simulink model "ATOM_simple_planning_simulator"  (R2026a)
settings: Solver=ode4  StopTime=100  FixedStep=0.01
StopFcn:
  | % Put every new figure in the same MATLAB Figures window as a docked tab.
  | set(groot, 'defaultFigureWindowStyle', 'docked');
  | 
  | if exist('costmap_active', 'var') && ...
  |     exist('vehicle', 'var') && ...
  |     exist('parking_path', 'var') && ...
  |     ~isempty(parking_path)
  | 
  |      plotPlan(costmap_active, vehicle, parking_path);
  | 
  |  else
  | 
  |      warning('No valid parking path is available for plotting.');
  | 
  |  end
  | 
  |  PlotControllerReferences( ...
  |      out.controller_reference_log);
  | 
  |  PlotControllerTracking( ...
  |      out.controller_tracking_log);
  | 
model workspace (MAT data in the model file):
  vehicle.param.wheel_radius = 0.313
  vehicle.param.wheel_width = 0.235
  vehicle.param.wheel_base = 2
  vehicle.param.wheel_tread = 1.9
  vehicle.param.front_overhang = 0.46
  vehicle.param.rear_overhang = 0.46
  vehicle.param.left_overhang = 0.128
  vehicle.param.right_overhang = 0.128
  vehicle.param.vehicle_height = 1.8
  vehicle.param.max_steer_angle = 0.7
  vehicle.sim.vehicle_model_type = "DELAY_STEER_ACC_GEARED"
  vehicle.sim.initialize_source = "INITIAL_POSE_TOPIC"
  vehicle.sim.timer_sampling_time_ms = 25
  vehicle.sim.add_measurement_noise = 0
  vehicle.sim.vel_lim = 50
  vehicle.sim.vel_rate_lim = 7
  vehicle.sim.steer_lim = 1
  vehicle.sim.steer_rate_lim = 5
  vehicle.sim.acc_time_delay = 0.1
  vehicle.sim.acc_time_constant = 0.1
  vehicle.sim.steer_time_delay = 0.24
  vehicle.sim.steer_time_constant = 0.27
  vehicle.sim.x_stddev = 0.0001
  vehicle.sim.y_stddev = 0.0001
  vehicle.sim.steer_dead_band = 0
  vehicle.sim.steer_bias = 0
  vehicle.sim.debug_acc_scaling_factor = 1
  vehicle.sim.debug_steer_scaling_factor = 1
undefined symbols (not defined in the file): delta_f_LUT, gain4WS_LUT, k_ref_LUT, kappa_gain_BP, Ki, Kp, lateral, longitudinal, planning_validator, rr_gain_BP, rr_LUT, stanley, velocity_smoother
libraries: slpidlib x1
(part 1 of 8)
settings Model: PacingRate=1000  Creator=andrea-ricetti  LastModifiedBy=husain5

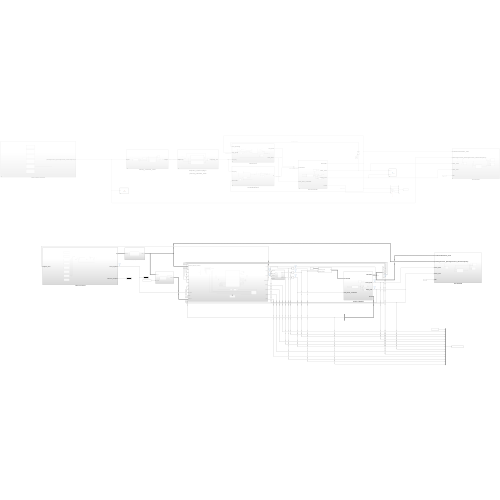
[thumbnail: Simulink's stored preview of the top-level diagram]
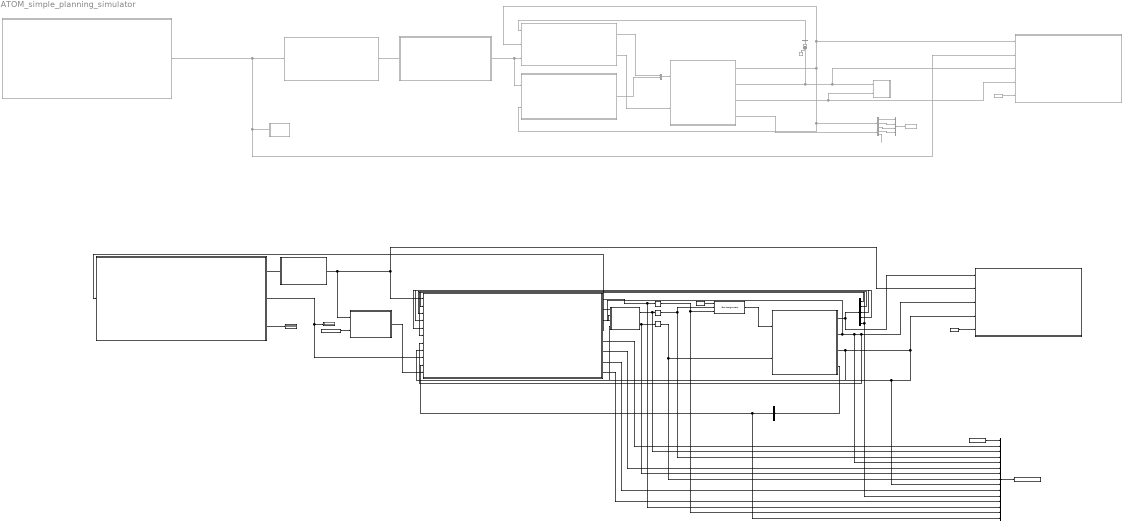
== system ATOM_simple_planning_simulator ==
  Add : Sum  Commented=on
  Bus Assignment2 : BusAssignment  AssignedSignals=lateral.steering_tire_angle,longitudinal.acceleration
  Bus Creator3 : BusCreator  Commented=on  Inputs=1  OutDataTypeStr=Bus: SteeringBus
      settings: InheritFromInputs=off
  Bus Selector : BusSelector  Commented=on  OutputSignals=pose.position.x,pose.position.y,twist.linear.x
  Bus Selector1 : BusSelector  Commented=on  OutputSignals=acceleration.linear.x,acceleration.linear.y
  Bus Selector5 : BusSelector  OutputSignals=pose.position.x,pose.position.y,pose.orientation.z,pose.orientation.w,twist.linear.x
  Bus Selector6 : BusSelector  OutputSignals=acceleration.linear.x
  Constant4 : Constant  Value=0  OutDataTypeStr=Bus: ControlCMDBus
  Constant5 : Constant  Value=vehicle.sim.steer_rate_lim
  Digital Clock2 : DigitalClock  SampleTime=0.04
  Display4 : Display
  Display5 : Display
  From Workspace1 : FromWorkspace  Commented=on  VariableName=veh
  From Workspace3 : FromWorkspace  VariableName=veh
  Lane Follower Scenario : Subsystem  Commented=on
  Lateral run() : Subsystem  Commented=on
  Lateral&Longitudinal_ControlCommand : BusCreator  Commented=on  Inputs=2  OutDataTypeStr=Bus: ControlCMDBus
      settings: InheritFromInputs=off
  LongitudinalRun() : Subsystem  Commented=on
  Mux : Mux  Commented=on
  Mux3 : Mux  Inputs=15
  Parking Scenario2 : Subsystem
  Plot demanded trajectory : MATLAB Function  Commented=on  TreatAsAtomicUnit=on
  Plot front/rear steer status : MATLAB Function  Commented=on  TreatAsAtomicUnit=on
  Plot vehicle : Subsystem  Commented=on
  Plot vehicle3 : Subsystem
  Subsystem2 : Subsystem
  To Workspace : ToWorkspace  Commented=on  VariableName=veh_log  SampleTime=0.05
  To Workspace3 : ToWorkspace  VariableName=controller_tracking_log  SaveFormat=Timeseries  SampleTime=-1
  Transport Delay6 : TransportDelay  DelayTime=vehicle.sim.acc_time_delay
  Transport Delay7 : TransportDelay  DelayTime=vehicle.sim.steer_time_delay
  Transport Delay8 : TransportDelay  DelayTime=vehicle.sim.steer_time_delay
  Vehicle Model : Subsystem  Commented=on
  Vehicle_Model2 : Subsystem
  parking_velocity_smoother2 : Subsystem
  steer_bias : Constant  Commented=on  Value=0
  steeringRatetoAngle2 : Subsystem
  time_parameterization2 : Subsystem
  trajectory_checker plugin - planning_validator_node : Subsystem  Commented=on
  velocity_smoother_node : Subsystem  Commented=on
  wires:
  LongitudinalRun()/1(Out1) -> Lateral&Longitudinal_ControlCommand/2  "LongitudinalCommand"
  Lateral&Longitudinal_ControlCommand/1 -> Vehicle Model/1(command)
  Vehicle Model/1(kinematic) -> LongitudinalRun()/2(kinematic), Bus Selector/1, Plot vehicle/1(localization/kinematic_state), Lateral run()/2(ego_pose)  "/localization/kinematic_state"
  Vehicle Model/3(steer_rear) -> Plot front/rear steer status/2(rear_steer), Plot vehicle/4(steer_rear)
  Vehicle Model/4(accel) -> Bus Selector1/1  "/localization/acceleration"
  trajectory_checker plugin - planning_validator_node/1(trajectory_out) -> LongitudinalRun()/1(ref_traj), Lateral run()/3(ref_traj)  "/planning/trajectory"
  Bus Creator3/1 -> Lateral run()/1(curr_steering)  "/vehicle/status/steering_status"
  Add/1 -> Bus Creator3/1
  steer_bias/1 -> Add/1
  Vehicle Model/2(steer_front) -> Add/2, Plot vehicle/3(steer_front), Plot front/rear steer status/1(front_steer)
  From Workspace1/1 -> Plot vehicle/5(veh)
  Lateral run()/1(ctrl_cmd) -> Lateral&Longitudinal_ControlCommand/1  "LateralCommand"
  velocity_smoother_node/1(output) -> trajectory_checker plugin - planning_validator_node/1(trajectory)  "/planning/scenario_planning/scenario_selector/trajectory"
  Bus Selector/1 -> Mux/1  "<x>"
  Bus Selector/2 -> Mux/2  "<y>"
  Bus Selector/3 -> Mux/3  "<x>"
  Bus Selector1/1 -> Mux/4  "<x>"
  Mux/1 -> To Workspace/1
  Lateral run()/2(rear_steer) -> Vehicle Model/2(rear_steer_commanf)
  Bus Selector1/2 -> ?  "<y>"
  Lane Follower Scenario/1(planning/scenario_planning/scenario_selector/trajectory4) -> Plot vehicle/2(planning/scenario_planning/scenario_selector/trajectory), Plot demanded trajectory/1(traj), velocity_smoother_node/1(input)
  Transport Delay8/1 -> Vehicle_Model2/2(rear_steer_commanf), Mux3/8
  Transport Delay6/1 -> Mux3/14, Bus Assignment2/3
  Vehicle_Model2/4(accel) -> Bus Selector6/1  "/localization/acceleration"
  Vehicle_Model2/1(kinematic) -> Plot vehicle3/1(localization/kinematic_state), Bus Selector5/1  "/localization/kinematic_state"
  Vehicle_Model2/3(steer_rear) -> steeringRatetoAngle2/4(dr_measured), Mux3/9, Subsystem2/8(dr), Plot vehicle3/4(steer_rear)
  Subsystem2/3(dr_cmd) -> steeringRatetoAngle2/2(dr_rate_cmd)
  Bus Selector5/2 -> Subsystem2/3(Y)  "<y>"
  steeringRatetoAngle2/1(df_angle_cmd) -> Mux3/3, Transport Delay7/1
  Subsystem2/2(df_cmd) -> steeringRatetoAngle2/1(df_rate_cmd)
  Parking Scenario2/1(traj) -> parking_velocity_smoother2/1(trajectory_in)
  Bus Selector5/5 -> Mux3/11, Subsystem2/6(vx)  "<x>"
  Mux3/1 -> To Workspace3/1
  time_parameterization2/1(reference_out) -> Subsystem2/11(reference_out)
  parking_velocity_smoother2/1(trajectory_out) -> time_parameterization2/1(trajectory_in), Subsystem2/1(planning/scenario_planning/scenario_selector/trajectory), Plot vehicle3/2(planning/scenario_planning/scenario_selector/trajectory)
  Digital Clock2/1 -> Mux3/1
  Bus Selector5/3 -> Subsystem2/4(qz)  "<z>"
  Bus Selector5/4 -> Subsystem2/5(qw)  "<w>"
  Constant5/1 -> time_parameterization2/2(steer_rate_limit)
  Subsystem2/4(segment_done) -> Parking Scenario2/1(segment_done)
  From Workspace3/1 -> Plot vehicle3/5(veh)
  Subsystem2/7(v_ref_out) -> Mux3/10
  Subsystem2/6(dr_ref_out) -> Mux3/6
  Subsystem2/5(df_ref_out) -> Mux3/2
  Bus Selector5/1 -> Subsystem2/2(X)  "<x>"
  Parking Scenario2/3(maneuver_complete) -> Display5/1
  steeringRatetoAngle2/2(dr_angle_cmd) -> Transport Delay8/1, Mux3/7
  Vehicle_Model2/2(steer_front) -> steeringRatetoAngle2/3(df_measured), Mux3/5, Subsystem2/7(df), Plot vehicle3/3(steer_front)
  Parking Scenario2/2(active_segment) -> Subsystem2/9(active_segment), Display4/1
  Bus Assignment2/1 -> Vehicle_Model2/1(command)
  Constant4/1 -> Bus Assignment2/1
  Subsystem2/8(a_ref_out) -> Mux3/12
  Bus Selector6/1 -> Subsystem2/10(ax_meas), Mux3/15  "<x>"
  Transport Delay7/1 -> Bus Assignment2/2, Mux3/4
  Subsystem2/1("a_cmd ") -> Transport Delay6/1, Mux3/13

== system ATOM_simple_planning_simulator/Lane Follower Scenario ==
  Demanded trajectory generation: 90° left turn : Subsystem
  Demanded trajectory generation: 90° left turn critical for 2WS --> R = 2.5 m : Subsystem
  Demanded trajectory generation: Serpentine : Subsystem
  Demanded trajectory generation: Sinusoid 50m wavelength : Subsystem
  Demanded trajectory generation: smooth Parabola : Subsystem
  Straight trajectory : Subsystem
  planning/scenario_planning/scenario_selector/trajectory4 : Outport
  wires:
  Demanded trajectory generation: Sinusoid 50m wavelength/1(traj) -> ?  "/planning/scenario_planning/scenario_selector/trajectory"
  Demanded trajectory generation: smooth Parabola/1(traj) -> ?  "/planning/scenario_planning/scenario_selector/trajectory"
  Straight trajectory/1(traj) -> ?  "/planning/scenario_planning/scenario_selector/trajectory"
  Demanded trajectory generation: 90° left turn/1(traj) -> ?  "/planning/scenario_planning/scenario_selector/trajectory"
  Demanded trajectory generation: Serpentine/1(traj) -> ?  "/planning/scenario_planning/scenario_selector/trajectory"
  Demanded trajectory generation: 90° left turn critical for 2WS --> R = 2.5 m/1(traj) -> planning/scenario_planning/scenario_selector/trajectory4/1  "/planning/scenario_planning/scenario_selector/trajectory"

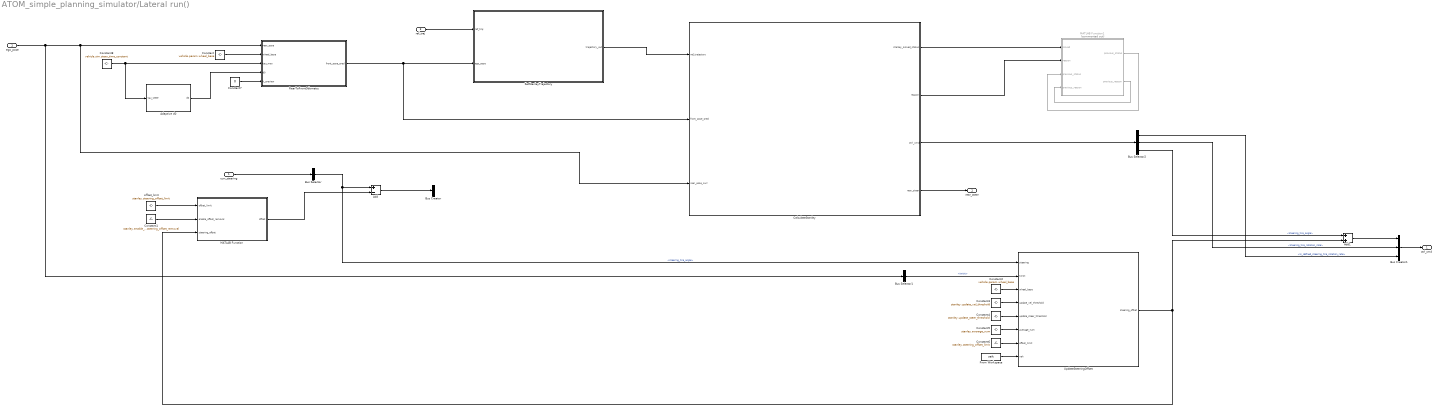
== system ATOM_simple_planning_simulator/Lateral run() ==
  curr_steering : Inport
  ego_pose : Inport  Port=2
  ref_traj : Inport  Port=3
  Adaptive d0 : MATLAB Function  TreatAsAtomicUnit=on
  Add : Sum  Inputs=+-
  Add1 : Sum
  Bus Creator : BusCreator  Inputs=1  OutDataTypeStr=Bus: SteeringBus
      settings: InheritFromInputs=off
  Bus Creator1 : BusCreator  Inputs=3  OutDataTypeStr=Bus: LateralBus
      settings: InheritFromInputs=off
  Bus Selector : BusSelector  OutputSignals=steering_tire_angle
  Bus Selector1 : BusSelector  OutputSignals=twist
  Bus Selector2 : BusSelector  OutputSignals=is_defined_steering_tire_rotation_rate,steering_tire_rotation_rate,steering_tire_angle
  CalculateStanley : Subsystem
  Constant : Constant  Value=vehicle.param.wheel_base
  Constant1 : Constant  Value=stanley.enable_auto_steering_offset_removal
  Constant2 : Constant  Value=vehicle.param.wheel_base
  Constant3 : Constant  Value=stanley.update_vel_threshold
  Constant4 : Constant  Value=stanley.update_steer_threshold
  Constant5 : Constant  Value=stanley.average_num
  Constant6 : Constant  Value=stanley.steering_offset_limit
  Constant7 : Constant  Value=0
  Constant8 : Constant  Value=vehicle.sim.steer_time_constant
  From Workspace : FromWorkspace  VariableName=veh
  MATLAB Function : MATLAB Function  TreatAsAtomicUnit=on
  MATLAB Function1 : MATLAB Function  Commented=on  TreatAsAtomicUnit=on
  RearToFrontOdometry : MATLAB Function  TreatAsAtomicUnit=on
  SetStanleyTrajectory : Subsystem
  UpdateSteeringOffset : MATLAB Function  TreatAsAtomicUnit=on
  offset_limit : Constant  Value=stanley.steering_offset_limit
  ctrl_cmd : Outport
  rear_steer : Outport  Port=2
  wires:
  ego_pose/1 -> Bus Selector1/1, CalculateStanley/3(rear_pose_curr), RearToFrontOdometry/1(rear_pose)
  Constant/1 -> RearToFrontOdometry/2(wheel_base)
  RearToFrontOdometry/1(front_pose_pred) -> CalculateStanley/2(front_pose_pred), SetStanleyTrajectory/2(ego_pose)
  curr_steering/1 -> Bus Selector/1
  offset_limit/1 -> MATLAB Function/1(offset_limit)
  Constant1/1 -> MATLAB Function/2(enable_offset_removal)
  Add/1 -> Bus Creator/1
  Bus Selector/1 -> UpdateSteeringOffset/1(steering), Add/1  "<steering_tire_angle>"
  ref_traj/1 -> SetStanleyTrajectory/1(ref_traj)
  SetStanleyTrajectory/1(trajectory_out) -> CalculateStanley/1(ref_trajectory)
  CalculateStanley/1(stanley_solved_status) -> MATLAB Function1/1(solved)
  CalculateStanley/2(reason) -> MATLAB Function1/2(reason)
  MATLAB Function1/2(previous_reason) -> MATLAB Function1/4("previous_reason ")
  MATLAB Function1/1(previous_status) -> MATLAB Function1/3("previous_status ")
  Bus Selector1/1 -> UpdateSteeringOffset/2(twist)  "<twist>"
  Constant2/1 -> UpdateSteeringOffset/3(wheel_base)
  Constant3/1 -> UpdateSteeringOffset/4(update_vel_threshold)
  Constant5/1 -> UpdateSteeringOffset/6(average_num)
  Constant4/1 -> UpdateSteeringOffset/5(update_steer_threshold)
  Constant6/1 -> UpdateSteeringOffset/7(offset_limit)
  From Workspace/1 -> UpdateSteeringOffset/8(veh)
  CalculateStanley/3(ctrl_cmd) -> Bus Selector2/1
  Bus Selector2/3 -> Add1/1  "<steering_tire_angle>"
  Add1/1 -> Bus Creator1/1
  Bus Selector2/1 -> Bus Creator1/3  "<is_defined_steering_tire_rotation_rate>"
  Bus Selector2/2 -> Bus Creator1/2  "<steering_tire_rotation_rate>"
  Bus Creator1/1 -> ctrl_cmd/1
  MATLAB Function/1(offset) -> Add/2
  UpdateSteeringOffset/1(steering_offset) -> MATLAB Function/3(steering_offset), Add1/2
  Constant8/1 -> Adaptive d0/1(tau_steer), RearToFrontOdometry/3(tau_max)
  Adaptive d0/1(d0) -> RearToFrontOdometry/4(d0)
  Constant7/1 -> RearToFrontOdometry/5(k_preview)
  CalculateStanley/4(rear_steer) -> rear_steer/1

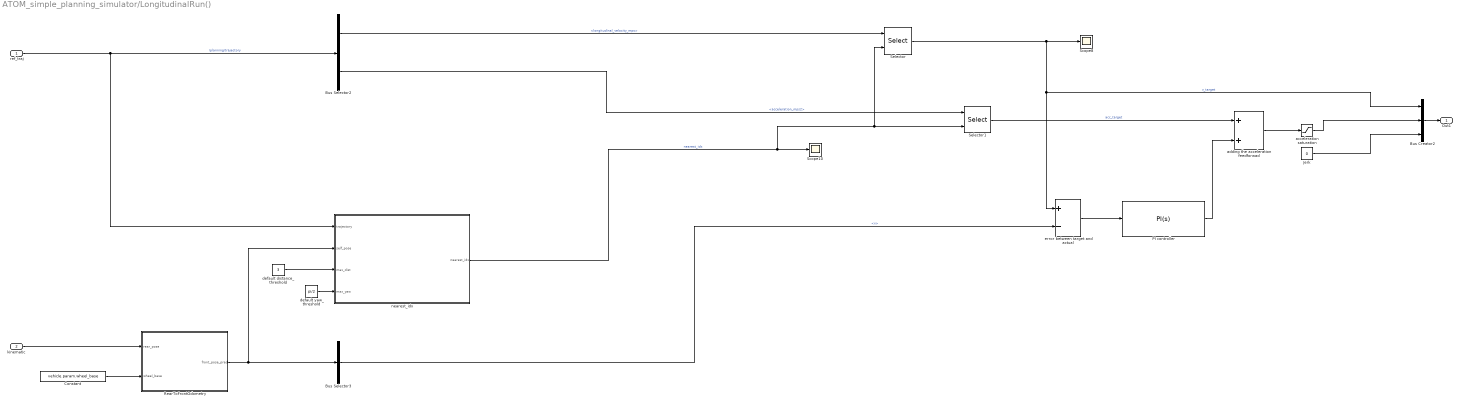
== system ATOM_simple_planning_simulator/LongitudinalRun() ==
  ref_traj : Inport
  kinematic : Inport  Port=2
  Bus Creator2 : BusCreator  Inputs=3  OutDataTypeStr=Bus: LongitudinalBus
      settings: InheritFromInputs=off
  Bus Selector2 : BusSelector  OutputSignals=longitudinal_velocity_mps,acceleration_mps2
  Bus Selector3 : BusSelector  OutputSignals=twist.linear.x
  Constant : Constant  Value=vehicle.param.wheel_base
  Jerk : Constant  Value=0
  PI controller : slpidlib/PID Controller  Controller=PI  Form=Parallel  TimeDomain=Continuous-time  UseExternalTs=off  SampleTime=-1  IntegratorMethod=Forward Euler  FilterMethod=Forward Euler  ControllerParametersSource=internal  P=Kp  I=Ki  UseKiTs=off  D=0  UseExternalDerivativeSource=off  N=100  UseFilter=on  TunerSelectOption=Transfer Function Based (PID Tuner App)  InitialConditionSource=internal  InitialConditionForIntegrator=0  InitialConditionForFilter=0  DifferentiatorICPrevScaledInput=0  ExternalReset=none  TrackingMode=off  Kt=1  LimitOutput=on  SatLimitsSource=internal  UpperSaturationLimit=+7.0  LowerSaturationLimit=-7.0  LinearizeAsGain=on  AntiWindupMode=clamping  Kb=1  LimitIntegrator=off  UpperIntegratorSaturationLimit=inf  LowerIntegratorSaturationLimit=-inf  POutMin=[]  POutMax=[]  IOutMin=[]  IOutMax=[]  DOutMin=[]  DOutMax=[]  NOutMin=[]  NOutMax=[]  SumOutMin=[]  SumOutMax=[]  SaturationOutMin=[]  SaturationOutMax=[]  PParamMin=[]  PParamMax=[]  IParamMin=[]  IParamMax=[]  DParamMin=[]  DParamMax=[]  NParamMin=[]  NParamMax=[]  KbParamMin=[]  KbParamMax=[]  KtParamMin=[]  KtParamMax=[]  KbOutMin=[]  KbOutMax=[]  KtOutMin=[]  KtOutMax=[]  IntegratorOutMin=[]  IntegratorOutMax=[]  FilterOutMin=[]  FilterOutMax=[]  SumI1OutMin=[]  SumI1OutMax=[]  SumI2OutMin=[]  SumI2OutMax=[]  SumI3OutMin=[]  SumI3OutMax=[]  SumI4OutMin=[]  SumI4OutMax=[]  SumDOutMin=[]  SumDOutMax=[]  DifferentiatorOutMin=[]  DifferentiatorOutMax=[]  FilterDiffOutCoefMin=[]  FilterDiffOutCoefMax=[]  ReciprocalOutMin=[]  ReciprocalOutMax=[]  SumDenOutMin=[]  SumDenOutMax=[]  SumNumOutMin=[]  SumNumOutMax=[]  DivideOutMin=[]  DivideOutMax=[]  UdiffTsProdOutMin=[]  UdiffTsProdOutMax=[]  NTsProdOutMin=[]  NTsProdOutMax=[]  UintegralTsProdOutMin=[]  UintegralTsProdOutMax=[]  UngainTsProdOutMin=[]  UngainTsProdOutMax=[]  ClampingZeroOutDataTypeStr=Inherit: Inherit via back propagation  ClampingZeroOutMin=[]  ClampingZeroOutMax=[]  FilterDenConstantOutDataTypeStr=Inherit: Inherit via back propagation  FilterDenConstantOutMin=[]  FilterDenConstantOutMax=[]  PCopyOutDataTypeStr=Inherit: Inherit via back propagation  PCopyOutMin=[]  PCopyOutMax=[]  NCopyOutDataTypeStr=Inherit: Inherit via back propagation  NCopyOutMin=[]  NCopyOutMax=[]  IntegratorContinuousStateAttributes=''  IntegratorStateMustResolveToSignalObject=off  IntegratorRTWStateStorageClass=Auto  FilterContinuousStateAttributes=''  FilterStateMustResolveToSignalObject=off  FilterRTWStateStorageClass=Auto  ParallelPVariant=InternalParameters  IdealPVariant=Disabled  IVariant=InternalParameters  DVariant=Disabled  IntegratorVariant=Continuous  SatVariant=Enabled  AWVariant=ContClampingParallel  PCopyVariant=Disabled  TRVariant=Disabled  FdbkBlocksVariant=Forward  IdealPFdbkVariant=Disabled  SatFdbkVariant=Disabled  DerivativeFilterVariant=Disabled  NVariant=Disabled  NCopyVariant=Disabled_SignalSpec  FilterICVariant=Disabled  IntegratorICVariant=InternalICs  ExternalResetVariant=Disabled  TRSumVariant=Passthrough  SumFdbkVariant=Disabled  SumVariant=Sum_PI  TsampFilterVariant=InternalTs  TsampNgainVariant=Passthrough  TsampIntegralVariant=Disabled_SignalSpec  ExternalSaturationOutDataTypeStr=Inherit: Same as second input  DerivativeSourceVariant=Disabled  PreIntVariant=InternalPreInt
  RearToFrontOdometry : MATLAB Function  TreatAsAtomicUnit=on
  Scope10 : Scope
      settings: ActiveDisplayYMinimum=-3.3749999999999991  ActiveDisplayYMaximum=40.375  DataLoggingVariableName=ScopeData18
  Scope8 : Scope
      settings: ActiveDisplayYMinimum=0.37500000000000044  ActiveDisplayYMaximum=16.625  DataLoggingVariableName=ScopeData16
  Selector : Selector  IndexOptions=Index vector (port)  Indices=[1 3]  OutputSizes=1
  Selector1 : Selector  IndexOptions=Index vector (port)  Indices=[1 3]  OutputSizes=1
  acceleration saturation : Saturate  UpperLimit=velocity_smoother.max_acc  LowerLimit=velocity_smoother.min_acc
  adding the acceleration feedforwad : Sum
  default distance_threshold : Constant  Value=3
  default yaw_threshold : Constant  Value=pi/2
  error between target and actual : Sum  Inputs=+-
  nearest_idx : MATLAB Function  TreatAsAtomicUnit=on
  Out1 : Outport
  wires:
  Bus Creator2/1 -> Out1/1
  RearToFrontOdometry/1(front_pose_pred) -> Bus Selector3/1, nearest_idx/2(self_pose)
  ref_traj/1 -> Bus Selector2/1, nearest_idx/1(trajectory)  "/planning/trajectory"
  Bus Selector2/1 -> Selector/1  "<longitudinal_velocity_mps>"
  PI controller/1 -> adding the acceleration feedforwad/2
  Bus Selector2/2 -> Selector1/1  "<acceleration_mps2>"
  error between target and actual/1 -> PI controller/1
  Selector/1 -> error between target and actual/1, Bus Creator2/1, Scope8/1  "v_target"
  Jerk/1 -> Bus Creator2/3
  adding the acceleration feedforwad/1 -> acceleration saturation/1
  nearest_idx/1(nearest_idx) -> Scope10/1, Selector1/2, Selector/2  "nearest_idx"
  Selector1/1 -> adding the acceleration feedforwad/1  "acc_target"
  Bus Selector3/1 -> error between target and actual/2  "<x>"
  acceleration saturation/1 -> Bus Creator2/2
  Constant/1 -> RearToFrontOdometry/2(wheel_base)
  kinematic/1 -> RearToFrontOdometry/1(rear_pose)
  default distance_threshold/1 -> nearest_idx/3(max_dist)
  default yaw_threshold/1 -> nearest_idx/4(max_yaw)

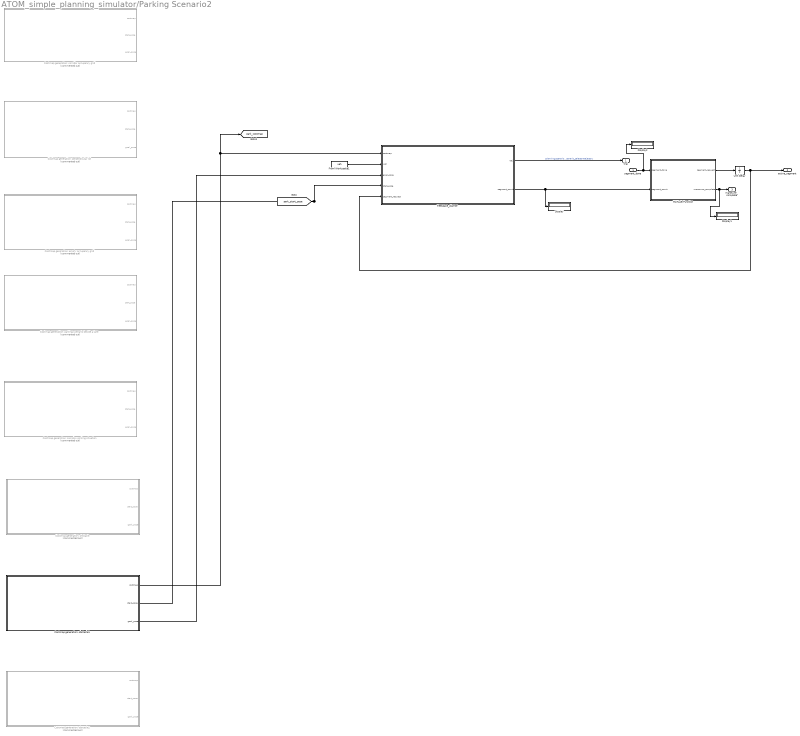
== system ATOM_simple_planning_simulator/Parking Scenario2 ==
  segment_done : Inport
  Costmap generation: complex parking situation : Subsystem  Commented=on
  Costmap generation: corridor occupancy grid : Subsystem  Commented=on
  Costmap generation: empty occupancy grid : Subsystem  Commented=on
  Costmap generation: obstacle : Subsystem  Commented=on
  Costmap generation: obstacle1 : Subsystem
  Costmap generation: obstacle2 : Subsystem  Commented=on
  Costmap generation: parking scenario beside a lane : Subsystem  Commented=on
  Costmap generation: perpendicular lot : Subsystem  Commented=on
  Display : Display
  Display1 : Display
  Display2 : Display
  From Workspace1 : FromWorkspace  VariableName=veh
  MATLAB Function : MATLAB Function  TreatAsAtomicUnit=on
  Unit Delay : UnitDelay  InitialCondition=1  SampleTime=0.04
  freespace_planner : Subsystem
  traj : Outport
  active_segment : Outport  Port=2
  maneuver_complete : Outport  Port=3
  tag scope: park_costmap=global, park_start_pose=global
  wires:
  Costmap generation: obstacle1/1(costmap) -> [park_costmap], freespace_planner/1(costmap)
  From Workspace1/1 -> freespace_planner/2(veh)
  Costmap generation: obstacle1/3(goal_pose) -> freespace_planner/3(goal_pose)
  Costmap generation: obstacle1/2(start_pose) -> freespace_planner/4(start_pose), [park_start_pose]
  freespace_planner/1(traj) -> traj/1  "/planning/scenario_planning/scenario_selector/trajectory"
  Unit Delay/1 -> freespace_planner/5(segment_request), active_segment/1
  freespace_planner/2(segment_count) -> Display/1, MATLAB Function/2(segment_count)
  segment_done/1 -> Display2/1, MATLAB Function/1(segment_done)
  MATLAB Function/1(segment_request) -> Unit Delay/1
  MATLAB Function/2(maneuver_complete) -> Display1/1, maneuver_complete/1

== system ATOM_simple_planning_simulator/Plot vehicle ==
  localization/kinematic_state : Inport
  planning/scenario_planning/scenario_selector/trajectory : Inport  Port=2
  steer_front : Inport  Port=3
  steer_rear : Inport  Port=4
  veh : Inport  Port=5
  Constant : Constant  Value=vehicle.param.wheel_base
  Plot Vehicle Rear reference frame : MATLAB Function  TreatAsAtomicUnit=on
  Plot vehicle Front reference frame : MATLAB Function  TreatAsAtomicUnit=on
  RearToFrontOdometry : MATLAB Function  TreatAsAtomicUnit=on
  SetStanleyTrajectory : Subsystem
  wires:
  steer_rear/1 -> Plot vehicle Front reference frame/3(steer_rear), Plot Vehicle Rear reference frame/3(steer_rear)
  veh/1 -> Plot vehicle Front reference frame/4(veh), Plot Vehicle Rear reference frame/4(veh)
  steer_front/1 -> Plot vehicle Front reference frame/2(steer_front), Plot Vehicle Rear reference frame/2(steer_front)
  Constant/1 -> RearToFrontOdometry/2(wheel_base)
  localization/kinematic_state/1 -> Plot Vehicle Rear reference frame/1(kinematic), RearToFrontOdometry/1(rear_pose)
  planning/scenario_planning/scenario_selector/trajectory/1 -> SetStanleyTrajectory/1(ref_traj), Plot Vehicle Rear reference frame/5(traj)
  RearToFrontOdometry/1(front_pose) -> SetStanleyTrajectory/2(ego_pose), Plot vehicle Front reference frame/1(kinematic)
  SetStanleyTrajectory/1(trajectory_out) -> Plot vehicle Front reference frame/5(traj)

== system ATOM_simple_planning_simulator/Plot vehicle3 ==
  localization/kinematic_state : Inport
  planning/scenario_planning/scenario_selector/trajectory : Inport  Port=2
  steer_front : Inport  Port=3
  steer_rear : Inport  Port=4
  veh : Inport  Port=5
  Constant : Constant  Value=vehicle.param.wheel_base
  Plot Vehicle Rear reference frame : MATLAB Function  TreatAsAtomicUnit=on
  Plot vehicle Front reference frame : MATLAB Function  TreatAsAtomicUnit=on
  RearToFrontOdometry : MATLAB Function  TreatAsAtomicUnit=on
  SetStanleyTrajectory : Subsystem
  wires:
  steer_rear/1 -> Plot vehicle Front reference frame/3(steer_rear), Plot Vehicle Rear reference frame/3(steer_rear)
  veh/1 -> Plot vehicle Front reference frame/4(veh), Plot Vehicle Rear reference frame/4(veh)
  steer_front/1 -> Plot Vehicle Rear reference frame/2(steer_front), Plot vehicle Front reference frame/2(steer_front)
  Constant/1 -> RearToFrontOdometry/2(wheel_base)
  localization/kinematic_state/1 -> Plot Vehicle Rear reference frame/1(kinematic), RearToFrontOdometry/1(rear_pose)
  planning/scenario_planning/scenario_selector/trajectory/1 -> SetStanleyTrajectory/1(ref_traj), Plot Vehicle Rear reference frame/5(traj)
  RearToFrontOdometry/1(front_pose) -> SetStanleyTrajectory/2(ego_pose), Plot vehicle Front reference frame/1(kinematic)
  SetStanleyTrajectory/1(trajectory_out) -> Plot vehicle Front reference frame/5(traj)
  [park_costmap] -> Plot Vehicle Rear reference frame/6(costmap)

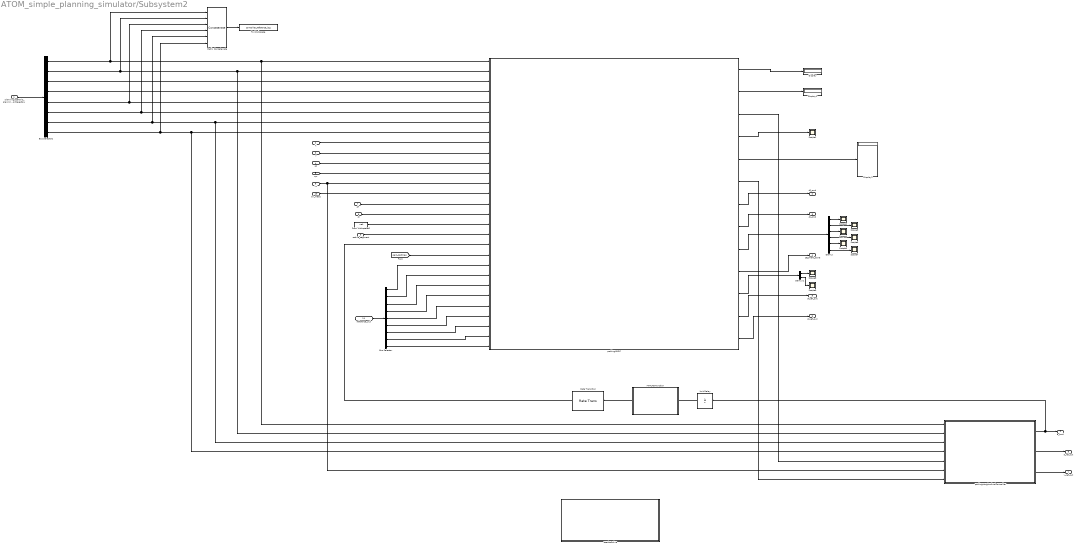
== system ATOM_simple_planning_simulator/Subsystem2 ==
  planning/scenario_planning/scenario_selector/trajectory : Inport
  X : Inport  Port=2
  Y : Inport  Port=3
  qz : Inport  Port=4
  qw : Inport  Port=5
  vx : Inport  Port=6
  df : Inport  Port=7
  dr : Inport  Port=8
  active_segment : Inport  Port=9
  ax_meas : Inport  Port=10
  reference_out : Inport  Port=11  OutDataTypeStr=Bus: ParkingReferenceBus  PortDimensions=1
  Bus Selector : BusSelector  OutputSignals=t_ref,s_ref,x_ref,y_ref,psi_ref,v_ref,a_ref,df_nom,dr_nom
  Bus Selector2 : BusSelector  OutputSignals=pose.position.x,pose.position.y,pose.orientation.qz,pose.orientation.qw,front_wheel_angle_rad,rear_wheel_angle_rad,longitudinal_velocity_mps,acceleration_mps2
  Demux : Demux  Outputs=6
  Demux1 : Demux  Outputs=2
  Display : Display
  Display1 : Display
  Display2 : Display
  From Workspace2 : FromWorkspace  VariableName=veh
  MATLAB Function : MATLAB Function  TreatAsAtomicUnit=on
  Matrix Concatenate : Concatenate  NumInputs=6  Mode=Multidimensional array  ConcatenateDimension=2
  Rate Transition : RateTransition  OutPortSampleTime=0.04
  Scope{1..9} (9 alike) : Scope
      Scope1 settings: ActiveDisplayYMinimum=-1  ActiveDisplayYMaximum=1  DataLoggingVariableName=ScopeData8
      Scope2 settings: ActiveDisplayYMinimum=-0.77251868208460861  ActiveDisplayYMaximum=0.080039739519414982  DataLoggingVariableName=ScopeData7
      Scope3 settings: ActiveDisplayYMinimum=-1  ActiveDisplayYMaximum=1  DataLoggingVariableName=ScopeData8
      Scope4 settings: ActiveDisplayYMinimum=-1  ActiveDisplayYMaximum=1  DataLoggingVariableName=ScopeData9
      Scope5 settings: ActiveDisplayYMinimum=-6.2499999999999982  ActiveDisplayYMaximum=56.25  DataLoggingVariableName=ScopeData10
      Scope6 settings: ActiveDisplayYMinimum=-1.2486948621003993  ActiveDisplayYMaximum=1.2498549846778222  DataLoggingVariableName=ScopeData11
      Scope7 settings: ActiveDisplayYMinimum=-0.87499999999999978  ActiveDisplayYMaximum=7.875  DataLoggingVariableName=ScopeData12
      Scope8 settings: ActiveDisplayYMinimum=-0.91973845897049766  ActiveDisplayYMaximum=8.3026771645702038  DataLoggingVariableName=ScopeData13
      Scope9 settings: ActiveDisplayYMinimum=-9.7701503022243354  ActiveDisplayYMaximum=73.160586445122291  DataLoggingVariableName=ScopeData14
  To Workspace : ToWorkspace  VariableName=controller_reference_log  SampleTime=-1
  Unit Delay : UnitDelay  SampleTime=0.04
  acadosSolve : Subsystem  TreatAsAtomicUnit=on
  parkingLongitudinalController : MATLAB Function  TreatAsAtomicUnit=on
  parkingNMPC : MATLAB Function  TreatAsAtomicUnit=on
  "a_cmd " : Outport
  df_cmd : Outport  Port=2
  dr_cmd : Outport  Port=3
  segment_done : Outport  Port=4
  df_ref_out : Outport  Port=5
  dr_ref_out : Outport  Port=6
  v_ref_out : Outport  Port=7
  a_ref_out : Outport  Port=8
  wires:
  Bus Selector2/5 -> Matrix Concatenate/3, parkingNMPC/5(tdf)  "<front_wheel_angle_rad>"
  parkingNMPC/2(max_q) -> Display1/1
  Bus Selector2/2 -> Matrix Concatenate/2, parkingLongitudinalController/2(ty), parkingNMPC/2(ty)  "<y>"
  Bus Selector2/4 -> parkingNMPC/4(tqw)  "<qw>"
  Bus Selector2/3 -> parkingNMPC/3(tqz)  "<qz>"
  Bus Selector2/1 -> parkingNMPC/1(tx), parkingLongitudinalController/1(tx), Matrix Concatenate/1  "<x>"
  parkingNMPC/1(path_length) -> Display/1
  Bus Selector2/6 -> Matrix Concatenate/4, parkingNMPC/6(tdr)  "<rear_wheel_angle_rad>"
  planning/scenario_planning/scenario_selector/trajectory/1 -> Bus Selector2/1
  X/1 -> parkingNMPC/9(X)
  Y/1 -> parkingNMPC/10(Y)
  parkingNMPC/3(s_now) -> parkingLongitudinalController/5(s_now)
  parkingNMPC/4(ey_now) -> Scope1/1
  qz/1 -> parkingNMPC/11(qz)
  qw/1 -> parkingNMPC/12(qw)
  vx/1 -> parkingNMPC/13(vx), parkingLongitudinalController/6(vx)
  df/1 -> parkingNMPC/15(df)
  dr/1 -> parkingNMPC/16(dr)
  parkingNMPC/5(x_now) -> Display2/1  "x_now"
  From Workspace2/1 -> parkingNMPC/17(veh)
  parkingNMPC/6(longitudinal_mode) -> parkingLongitudinalController/7(longitudinal_mode)
  parkingNMPC/7(df_rate_cmd) -> df_cmd/1
  parkingNMPC/8(dr_rate_cmd) -> dr_cmd/1
  parkingNMPC/9(nmpc_info) -> Demux/1
  Demux/1 -> Scope2/1
  Demux/2 -> Scope3/1
  Demux/3 -> Scope4/1
  Demux/4 -> Scope5/1
  Demux/5 -> Scope6/1
  Demux/6 -> Scope7/1
  Bus Selector2/7 -> Matrix Concatenate/5, parkingNMPC/7(tvx), parkingLongitudinalController/3(tvx)  "<longitudinal_velocity_mps>"
  parkingNMPC/10(segment_done) -> segment_done/1
  active_segment/1 -> parkingNMPC/18(active_segment)
  parkingNMPC/11(endpoint_error) -> Demux1/1
  Demux1/1 -> Scope8/1
  Demux1/2 -> Scope9/1
  Bus Selector2/8 -> Matrix Concatenate/6, parkingLongitudinalController/4(tax), parkingNMPC/8(tax)  "<acceleration_mps2>"
  ax_meas/1 -> parkingNMPC/14(ax_meas)
  MATLAB Function/1(a_cmd_history) -> Rate Transition/1
  parkingLongitudinalController/2(a_ref_out) -> a_ref_out/1
  [park_costmap] -> parkingNMPC/20(costmap)
  Matrix Concatenate/1 -> To Workspace/1
  parkingNMPC/12(df_ref_out) -> df_ref_out/1
  parkingNMPC/13(dr_ref_out) -> dr_ref_out/1
  parkingLongitudinalController/3(v_ref_out) -> v_ref_out/1
  reference_out/1 -> Bus Selector/1
  Bus Selector/1 -> parkingNMPC/21(t_ref)  "<t_ref>"
  Bus Selector/2 -> parkingNMPC/22(s_ref)  "<s_ref>"
  Bus Selector/3 -> parkingNMPC/23(x_ref)  "<x_ref>"
  Bus Selector/4 -> parkingNMPC/24(y_ref)  "<y_ref>"
  Bus Selector/5 -> parkingNMPC/25(psi_ref)  "<psi_ref>"
  Bus Selector/6 -> parkingNMPC/26(v_ref)  "<v_ref>"
  Bus Selector/7 -> parkingNMPC/27(a_ref)  "<a_ref>"
  Bus Selector/8 -> parkingNMPC/28(df_nom)  "<df_nom>"
  Bus Selector/9 -> parkingNMPC/29(dr_nom)  "<dr_nom>"
  Unit Delay/1 -> MATLAB Function/1(a_cmd_previous)
  Rate Transition/1 -> parkingNMPC/19(a_cmd_history)
  parkingLongitudinalController/1(a_cmd) -> Unit Delay/1, "a_cmd "/1

== system ATOM_simple_planning_simulator/Vehicle Model ==
  command : Inport
  rear_steer_commanf : Inport  Port=2
  From Workspace : FromWorkspace  VariableName=veh
  Vehicle Dynamics : Subsystem
  Vehicle internal state : Subsystem
      settings: PortSchema="{\"entries\":[{\"content\":{\"sides\":[{\"content\":{},\"type\":\"ConnectorPlacement.EquallySpacedRectSide\",\"uuid\":\"4a3566d2-c9ed-40f5-9383-803dea843249\"},{\"content\":{\"connectorIds\":[\"Out1\",\"Out2\"],\"side\":\"RIGHT\"},\"type\":\"ConnectorPlacement.EquallySpacedRectSide\",\"uuid\":\"38e6b545-4a7a-4953-bfc7-602e8f089057\"},{\"content\":{\"side\":\"TOP\"},\"type\":\"ConnectorPlacement.EquallySpacedRectSide\",\"uuid\":\"85394c7e-506c-43bc-a81e-512f61060685\"},{\"content\":{\"connectorIds\":[\"In1\"],\"side\":\"BOTTOM\"},\"type\":\"ConnectorPlacement.EquallySpacedRectSide\",\"uuid\":\"97da4b67-3c43-4e7d-b3d8-7f85e7f15c39\"}]},\"type\":\"ConnectorPlacement.EquallySpacedConnector\",\"uuid\":\"d0ddb274-13a9-46fc-8356-ac8c2bb4db82\"}],\"packageUris\":[\"http://schema.mathworks.com/mf0/Connector/R2020b\"],\"version\":\"1.0\"}"
  localization/acceleration function : MATLAB Function  TreatAsAtomicUnit=on
  localization/kinematic_state function : MATLAB Function  TreatAsAtomicUnit=on
  kinematic : Outport
  steer_front : Outport  Port=2
  steer_rear : Outport  Port=3
  accel : Outport  Port=4
  wires:
  From Workspace/1 -> localization/acceleration function/2(veh), localization/kinematic_state function/2(veh)
  Vehicle Dynamics/1(IntState) -> localization/kinematic_state function/1(state), localization/acceleration function/1(state), Vehicle internal state/1(IntState)
  Vehicle internal state/2(steer_rear) -> steer_rear/1
  command/1 -> Vehicle Dynamics/1(command)
  localization/kinematic_state function/1(kinematic) -> kinematic/1
  Vehicle internal state/1(steer_front) -> steer_front/1
  localization/acceleration function/1(accel) -> accel/1
  rear_steer_commanf/1 -> Vehicle Dynamics/2(rear_steer_command)

== system ATOM_simple_planning_simulator/Vehicle_Model2 ==
  command : Inport
  rear_steer_commanf : Inport  Port=2
  From Workspace : FromWorkspace  VariableName=veh
  Vehicle Dynamics : Subsystem
  Vehicle internal state : Subsystem
      settings: PortSchema="{\"entries\":[{\"content\":{\"sides\":[{\"content\":{},\"type\":\"ConnectorPlacement.EquallySpacedRectSide\",\"uuid\":\"4a3566d2-c9ed-40f5-9383-803dea843249\"},{\"content\":{\"connectorIds\":[\"Out1\",\"Out2\"],\"side\":\"RIGHT\"},\"type\":\"ConnectorPlacement.EquallySpacedRectSide\",\"uuid\":\"38e6b545-4a7a-4953-bfc7-602e8f089057\"},{\"content\":{\"side\":\"TOP\"},\"type\":\"ConnectorPlacement.EquallySpacedRectSide\",\"uuid\":\"85394c7e-506c-43bc-a81e-512f61060685\"},{\"content\":{\"connectorIds\":[\"In1\"],\"side\":\"BOTTOM\"},\"type\":\"ConnectorPlacement.EquallySpacedRectSide\",\"uuid\":\"97da4b67-3c43-4e7d-b3d8-7f85e7f15c39\"}]},\"type\":\"ConnectorPlacement.EquallySpacedConnector\",\"uuid\":\"d0ddb274-13a9-46fc-8356-ac8c2bb4db82\"}],\"packageUris\":[\"http://schema.mathworks.com/mf0/Connector/R2020b\"],\"version\":\"1.0\"}"
  localization/acceleration function : MATLAB Function  TreatAsAtomicUnit=on
  localization/kinematic_state function : MATLAB Function  TreatAsAtomicUnit=on
  kinematic : Outport
  steer_front : Outport  Port=2
  steer_rear : Outport  Port=3
  accel : Outport  Port=4
  wires:
  From Workspace/1 -> localization/acceleration function/2(veh), localization/kinematic_state function/2(veh)
  Vehicle Dynamics/1(IntState) -> localization/kinematic_state function/1(state), localization/acceleration function/1(state), Vehicle internal state/1(IntState)
  Vehicle internal state/2(steer_rear) -> steer_rear/1
  command/1 -> Vehicle Dynamics/1(command)
  localization/kinematic_state function/1(kinematic) -> kinematic/1
  Vehicle internal state/1(steer_front) -> steer_front/1
  localization/acceleration function/1(accel) -> accel/1
  rear_steer_commanf/1 -> Vehicle Dynamics/2(rear_steer_command)

== system ATOM_simple_planning_simulator/parking_velocity_smoother2 ==
  trajectory_in : Inport
  MATLAB Function : MATLAB Function  TreatAsAtomicUnit=on
  trajectory_out : Outport
  wires:
  trajectory_in/1 -> MATLAB Function/1(trajectory_in)
  MATLAB Function/1(trajectory_out) -> trajectory_out/1

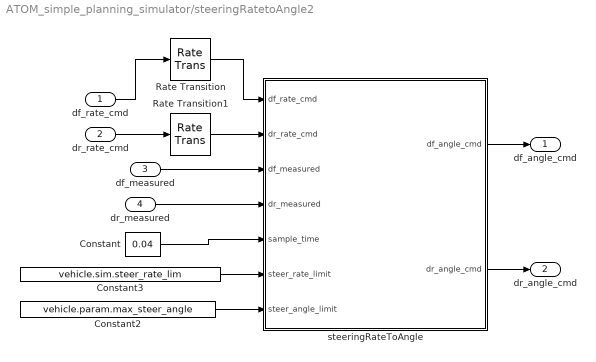
== system ATOM_simple_planning_simulator/steeringRatetoAngle2 ==
  df_rate_cmd : Inport
  dr_rate_cmd : Inport  Port=2
  df_measured : Inport  Port=3
  dr_measured : Inport  Port=4
  Constant : Constant  Value=0.04
  Constant2 : Constant  Value=vehicle.param.max_steer_angle
  Constant3 : Constant  Value=vehicle.sim.steer_rate_lim
  Rate Transition : RateTransition  OutPortSampleTime=0.04
  Rate Transition1 : RateTransition  OutPortSampleTime=0.04
  steeringRateToAngle : MATLAB Function  TreatAsAtomicUnit=on
  df_angle_cmd : Outport
  dr_angle_cmd : Outport  Port=2
  wires:
  steeringRateToAngle/2(dr_angle_cmd) -> dr_angle_cmd/1
  steeringRateToAngle/1(df_angle_cmd) -> df_angle_cmd/1
  dr_measured/1 -> steeringRateToAngle/4(dr_measured)
  df_measured/1 -> steeringRateToAngle/3(df_measured)
  dr_rate_cmd/1 -> Rate Transition1/1
  df_rate_cmd/1 -> Rate Transition/1
  Constant2/1 -> steeringRateToAngle/7(steer_angle_limit)
  Constant3/1 -> steeringRateToAngle/6(steer_rate_limit)
  Constant/1 -> steeringRateToAngle/5(sample_time)
  Rate Transition/1 -> steeringRateToAngle/1(df_rate_cmd)
  Rate Transition1/1 -> steeringRateToAngle/2(dr_rate_cmd)

== system ATOM_simple_planning_simulator/time_parameterization2 ==
  trajectory_in : Inport
  steer_rate_limit : Inport  Port=2
  Time parameterization : MATLAB Function  TreatAsAtomicUnit=on
  To Workspace : ToWorkspace  VariableName=time_parameterized_reference_log  SaveFormat=Timeseries  SampleTime=-1
  reference_out : Outport
  wires:
  trajectory_in/1 -> Time parameterization/1(trajectory_in)
  Time parameterization/1(reference_out) -> To Workspace/1, reference_out/1
  steer_rate_limit/1 -> Time parameterization/2(steer_rate_limit)

== system ATOM_simple_planning_simulator/trajectory_checker plugin - planning_validator_node ==
  trajectory : Inport
  From Workspace2 : FromWorkspace  VariableName=veh
  HandleInvalidTrajectory - handling_type == default (case 0) : MATLAB Function  TreatAsAtomicUnit=on
  check_valid_steering : Subsystem
  check_valid_steering_rate : Subsystem
  trajectory_out : Outport
  wires:
  From Workspace2/1 -> check_valid_steering_rate/2(veh), check_valid_steering/2(veh)
  trajectory/1 -> check_valid_steering_rate/1(trajectory), HandleInvalidTrajectory - handling_type == default (case 0)/1(trajectory_in), check_valid_steering/1(trajectory)
  check_valid_steering/1(is_valid_steering) -> HandleInvalidTrajectory - handling_type == default (case 0)/2(is_valid_steering)
  check_valid_steering_rate/1(is_valid_steering_rate) -> HandleInvalidTrajectory - handling_type == default (case 0)/3(is_valid_steering_rate)
  HandleInvalidTrajectory - handling_type == default (case 0)/1(trajectory_out) -> trajectory_out/1

== system ATOM_simple_planning_simulator/velocity_smoother_node ==
  input : Inport
  ApplyLateralAccelerationFilter - velocity_smoother node : Subsystem
  ApplySteeringRateLimit - velocity_smoother_node : Subsystem
  Bus Creator : BusCreator  Inputs=4
  Bus Selector : BusSelector  OutputSignals=longitudinal_velocity_mps,acceleration_mps2,pose.position.x,pose.position.y
  MATLAB Function : MATLAB Function  TreatAsAtomicUnit=on
  MATLAB Function1 : MATLAB Function  TreatAsAtomicUnit=on
  To Workspace : ToWorkspace  VariableName=log  SampleTime=0.05
  input_points_interval [m] : Constant  OutDataTypeStr=double
  use_resampling == false : Constant  Value=0  OutDataTypeStr=boolean
  output : Outport
  wires:
  input_points_interval [m]/1 -> ApplySteeringRateLimit - velocity_smoother_node/3(input_points_interval)
  ApplySteeringRateLimit - velocity_smoother_node/1(curvature) -> MATLAB Function1/3(curvature), ApplyLateralAccelerationFilter - velocity_smoother node/1(curvature), MATLAB Function/3(curvature)
  use_resampling == false/1 -> ApplySteeringRateLimit - velocity_smoother_node/2(use_resampling)
  input/1 -> ApplySteeringRateLimit - velocity_smoother_node/1(input From Trajecory topic --> TrajectoryPoints format), MATLAB Function/1(trajectory_input)
  ApplyLateralAccelerationFilter - velocity_smoother node/1(trajectory) -> MATLAB Function1/2(trajectory_output), Bus Selector/1, output/1
  ApplySteeringRateLimit - velocity_smoother_node/2(output) -> MATLAB Function/2(trajectory_output), MATLAB Function1/1(trajectory_input), ApplyLateralAccelerationFilter - velocity_smoother node/2("trajectory ")
  Bus Selector/1 -> Bus Creator/1  "<longitudinal_velocity_mps>"
  Bus Selector/2 -> Bus Creator/2  "<acceleration_mps2>"
  Bus Selector/3 -> Bus Creator/3  "<x>"
  Bus Selector/4 -> Bus Creator/4  "<y>"
  Bus Creator/1 -> To Workspace/1

== system ATOM_simple_planning_simulator/Lane Follower Scenario/Demanded trajectory generation: 90° left turn ==
  Bus Creator3 : BusCreator  Inputs=3  OutDataTypeStr=Bus: PointBusN
  Bus Creator4 : BusCreator  Inputs=4  OutDataTypeStr=Bus: QuaternionBusN
  Bus Creator5 : BusCreator  Inputs=2  OutDataTypeStr=Bus: PoseBusN
      settings: InheritFromInputs=off
  Bus Creator6 : BusCreator  Inputs=7  OutDataTypeStr=Bus: TrajectoryDataBus
      settings: InheritFromInputs=off
  Trajectory Generator: 90° left turn : MATLAB Function  TreatAsAtomicUnit=on
  traj : Outport
  wires:
  Bus Creator6/1 -> traj/1
  Bus Creator3/1 -> Bus Creator5/1
  Trajectory Generator: 90° left turn/13(rear_wheel_angle_rad) -> Bus Creator6/7
  Bus Creator5/1 -> Bus Creator6/1
  Trajectory Generator: 90° left turn/8(longitudinal_velocity_mps) -> Bus Creator6/2
  Trajectory Generator: 90° left turn/3(z) -> Bus Creator3/3
  Trajectory Generator: 90° left turn/4(qx) -> Bus Creator4/1
  Trajectory Generator: 90° left turn/9(lateral_velocity_mps) -> Bus Creator6/3
  Trajectory Generator: 90° left turn/10(acceleration_mps2) -> Bus Creator6/4
  Trajectory Generator: 90° left turn/5(qy) -> Bus Creator4/2
  Trajectory Generator: 90° left turn/1(x) -> Bus Creator3/1
  Trajectory Generator: 90° left turn/2(y) -> Bus Creator3/2
  Trajectory Generator: 90° left turn/7(qw) -> Bus Creator4/4
  Trajectory Generator: 90° left turn/6(qz) -> Bus Creator4/3
  Trajectory Generator: 90° left turn/12(front_wheel_angle_rad) -> Bus Creator6/6
  Bus Creator4/1 -> Bus Creator5/2
  Trajectory Generator: 90° left turn/11(heading_rate_rps) -> Bus Creator6/5

== system ATOM_simple_planning_simulator/Lane Follower Scenario/Demanded trajectory generation: 90° left turn critical for 2WS --> R = 2.5 m ==
  Bus Creator3 : BusCreator  Inputs=3  OutDataTypeStr=Bus: PointBusN
  Bus Creator4 : BusCreator  Inputs=4  OutDataTypeStr=Bus: QuaternionBusN
  Bus Creator5 : BusCreator  Inputs=2  OutDataTypeStr=Bus: PoseBusN
      settings: InheritFromInputs=off
  Bus Creator6 : BusCreator  Inputs=7  OutDataTypeStr=Bus: TrajectoryDataBus
      settings: InheritFromInputs=off
  Trajectory Generator: 90° left turn critical for 2WS : MATLAB Function  TreatAsAtomicUnit=on
  traj : Outport
  wires:
  Bus Creator6/1 -> traj/1
  Bus Creator3/1 -> Bus Creator5/1
  Trajectory Generator: 90° left turn critical for 2WS/13(rear_wheel_angle_rad) -> Bus Creator6/7
  Bus Creator5/1 -> Bus Creator6/1
  Trajectory Generator: 90° left turn critical for 2WS/8(longitudinal_velocity_mps) -> Bus Creator6/2
  Trajectory Generator: 90° left turn critical for 2WS/3(z) -> Bus Creator3/3
  Trajectory Generator: 90° left turn critical for 2WS/4(qx) -> Bus Creator4/1
  Trajectory Generator: 90° left turn critical for 2WS/9(lateral_velocity_mps) -> Bus Creator6/3
  Trajectory Generator: 90° left turn critical for 2WS/10(acceleration_mps2) -> Bus Creator6/4
  Trajectory Generator: 90° left turn critical for 2WS/5(qy) -> Bus Creator4/2
  Trajectory Generator: 90° left turn critical for 2WS/1(x) -> Bus Creator3/1
  Trajectory Generator: 90° left turn critical for 2WS/2(y) -> Bus Creator3/2
  Trajectory Generator: 90° left turn critical for 2WS/7(qw) -> Bus Creator4/4
  Trajectory Generator: 90° left turn critical for 2WS/6(qz) -> Bus Creator4/3
  Trajectory Generator: 90° left turn critical for 2WS/12(front_wheel_angle_rad) -> Bus Creator6/6
  Bus Creator4/1 -> Bus Creator5/2
  Trajectory Generator: 90° left turn critical for 2WS/11(heading_rate_rps) -> Bus Creator6/5

== system ATOM_simple_planning_simulator/Lane Follower Scenario/Demanded trajectory generation: Serpentine ==
  Bus Creator3 : BusCreator  Inputs=3  OutDataTypeStr=Bus: PointBusN
  Bus Creator4 : BusCreator  Inputs=4  OutDataTypeStr=Bus: QuaternionBusN
  Bus Creator5 : BusCreator  Inputs=2  OutDataTypeStr=Bus: PoseBusN
      settings: InheritFromInputs=off
  Bus Creator6 : BusCreator  Inputs=7  OutDataTypeStr=Bus: TrajectoryDataBus
      settings: InheritFromInputs=off
  Trajectory Generator: 90° left turn critical for 2WS : MATLAB Function  TreatAsAtomicUnit=on
  traj : Outport
  wires:
  Bus Creator6/1 -> traj/1
  Bus Creator3/1 -> Bus Creator5/1
  Trajectory Generator: 90° left turn critical for 2WS/13(rear_wheel_angle_rad) -> Bus Creator6/7
  Bus Creator5/1 -> Bus Creator6/1
  Trajectory Generator: 90° left turn critical for 2WS/8(longitudinal_velocity_mps) -> Bus Creator6/2
  Trajectory Generator: 90° left turn critical for 2WS/3(z) -> Bus Creator3/3
  Trajectory Generator: 90° left turn critical for 2WS/4(qx) -> Bus Creator4/1
  Trajectory Generator: 90° left turn critical for 2WS/9(lateral_velocity_mps) -> Bus Creator6/3
  Trajectory Generator: 90° left turn critical for 2WS/10(acceleration_mps2) -> Bus Creator6/4
  Trajectory Generator: 90° left turn critical for 2WS/5(qy) -> Bus Creator4/2
  Trajectory Generator: 90° left turn critical for 2WS/1(x) -> Bus Creator3/1
  Trajectory Generator: 90° left turn critical for 2WS/2(y) -> Bus Creator3/2
  Trajectory Generator: 90° left turn critical for 2WS/7(qw) -> Bus Creator4/4
  Trajectory Generator: 90° left turn critical for 2WS/6(qz) -> Bus Creator4/3
  Trajectory Generator: 90° left turn critical for 2WS/12(front_wheel_angle_rad) -> Bus Creator6/6
  Bus Creator4/1 -> Bus Creator5/2
  Trajectory Generator: 90° left turn critical for 2WS/11(heading_rate_rps) -> Bus Creator6/5

== system ATOM_simple_planning_simulator/Lane Follower Scenario/Demanded trajectory generation: Sinusoid 50m wavelength ==
  Bus Creator3 : BusCreator  Inputs=3  OutDataTypeStr=Bus: PointBusN
  Bus Creator4 : BusCreator  Inputs=4  OutDataTypeStr=Bus: QuaternionBusN
  Bus Creator5 : BusCreator  Inputs=2  OutDataTypeStr=Bus: PoseBusN
      settings: InheritFromInputs=off
  Bus Creator6 : BusCreator  Inputs=7  OutDataTypeStr=Bus: TrajectoryDataBus
      settings: InheritFromInputs=off
  Trajectory Generator: sinusoid : MATLAB Function  TreatAsAtomicUnit=on
  traj : Outport
  wires:
  Bus Creator6/1 -> traj/1
  Bus Creator3/1 -> Bus Creator5/1
  Trajectory Generator: sinusoid/13(rear_wheel_angle_rad) -> Bus Creator6/7
  Bus Creator5/1 -> Bus Creator6/1
  Trajectory Generator: sinusoid/8(longitudinal_velocity_mps) -> Bus Creator6/2
  Trajectory Generator: sinusoid/3(z) -> Bus Creator3/3
  Trajectory Generator: sinusoid/4(qx) -> Bus Creator4/1
  Trajectory Generator: sinusoid/9(lateral_velocity_mps) -> Bus Creator6/3
  Trajectory Generator: sinusoid/10(acceleration_mps2) -> Bus Creator6/4
  Trajectory Generator: sinusoid/5(qy) -> Bus Creator4/2
  Trajectory Generator: sinusoid/1(x) -> Bus Creator3/1
  Trajectory Generator: sinusoid/2(y) -> Bus Creator3/2
  Trajectory Generator: sinusoid/7(qw) -> Bus Creator4/4
  Trajectory Generator: sinusoid/6(qz) -> Bus Creator4/3
  Trajectory Generator: sinusoid/12(front_wheel_angle_rad) -> Bus Creator6/6
  Bus Creator4/1 -> Bus Creator5/2
  Trajectory Generator: sinusoid/11(heading_rate_rps) -> Bus Creator6/5

== system ATOM_simple_planning_simulator/Lane Follower Scenario/Demanded trajectory generation: smooth Parabola ==
  Bus Creator3 : BusCreator  Inputs=3  OutDataTypeStr=Bus: PointBusN
  Bus Creator4 : BusCreator  Inputs=4  OutDataTypeStr=Bus: QuaternionBusN
  Bus Creator5 : BusCreator  Inputs=2  OutDataTypeStr=Bus: PoseBusN
      settings: InheritFromInputs=off
  Bus Creator6 : BusCreator  Inputs=7  OutDataTypeStr=Bus: TrajectoryDataBus
      settings: InheritFromInputs=off
  Smoothed Parabola trajectory : MATLAB Function  TreatAsAtomicUnit=on
  traj : Outport
  wires:
  Smoothed Parabola trajectory/5(qy) -> Bus Creator4/2
  Smoothed Parabola trajectory/6(qz) -> Bus Creator4/3
  Smoothed Parabola trajectory/11(heading_rate_rps) -> Bus Creator6/5
  Bus Creator5/1 -> Bus Creator6/1
  Bus Creator6/1 -> traj/1
  Smoothed Parabola trajectory/3(z) -> Bus Creator3/3
  Bus Creator4/1 -> Bus Creator5/2
  Smoothed Parabola trajectory/8(longitudinal_velocity_mps) -> Bus Creator6/2
  Smoothed Parabola trajectory/4(qx) -> Bus Creator4/1
  Smoothed Parabola trajectory/13(rear_wheel_angle_rad) -> Bus Creator6/7
  Smoothed Parabola trajectory/7(qw) -> Bus Creator4/4
  Smoothed Parabola trajectory/1(x) -> Bus Creator3/1
  Smoothed Parabola trajectory/2(y) -> Bus Creator3/2
  Bus Creator3/1 -> Bus Creator5/1
  Smoothed Parabola trajectory/12(front_wheel_angle_rad) -> Bus Creator6/6
  Smoothed Parabola trajectory/10(acceleration_mps2) -> Bus Creator6/4
  Smoothed Parabola trajectory/9(lateral_velocity_mps) -> Bus Creator6/3

== system ATOM_simple_planning_simulator/Lane Follower Scenario/Straight trajectory ==
  Bus Creator3 : BusCreator  Inputs=3  OutDataTypeStr=Bus: PointBusN
  Bus Creator4 : BusCreator  Inputs=4  OutDataTypeStr=Bus: QuaternionBusN
  Bus Creator5 : BusCreator  Inputs=2  OutDataTypeStr=Bus: PoseBusN
      settings: InheritFromInputs=off
  Bus Creator6 : BusCreator  Inputs=7  OutDataTypeStr=Bus: TrajectoryDataBus
      settings: InheritFromInputs=off
  Trajectory Generator: straight : MATLAB Function  TreatAsAtomicUnit=on
  traj : Outport
  wires:
  Bus Creator6/1 -> traj/1
  Bus Creator3/1 -> Bus Creator5/1
  Trajectory Generator: straight/13(rear_wheel_angle_rad) -> Bus Creator6/7
  Bus Creator5/1 -> Bus Creator6/1
  Trajectory Generator: straight/8(longitudinal_velocity_mps) -> Bus Creator6/2
  Trajectory Generator: straight/3(z) -> Bus Creator3/3
  Trajectory Generator: straight/4(qx) -> Bus Creator4/1
  Trajectory Generator: straight/9(lateral_velocity_mps) -> Bus Creator6/3
  Trajectory Generator: straight/10(acceleration_mps2) -> Bus Creator6/4
  Trajectory Generator: straight/5(qy) -> Bus Creator4/2
  Trajectory Generator: straight/1(x) -> Bus Creator3/1
  Trajectory Generator: straight/2(y) -> Bus Creator3/2
  Trajectory Generator: straight/7(qw) -> Bus Creator4/4
  Trajectory Generator: straight/6(qz) -> Bus Creator4/3
  Trajectory Generator: straight/12(front_wheel_angle_rad) -> Bus Creator6/6
  Bus Creator4/1 -> Bus Creator5/2
  Trajectory Generator: straight/11(heading_rate_rps) -> Bus Creator6/5

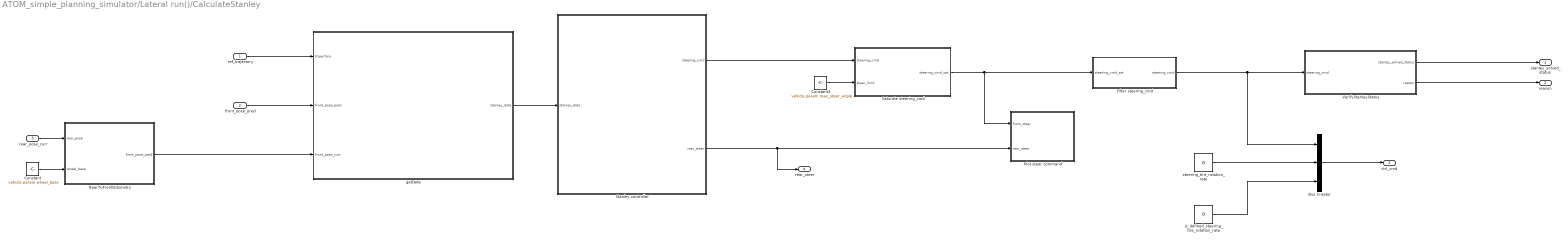
== system ATOM_simple_planning_simulator/Lateral run()/CalculateStanley ==
  ref_trajectory : Inport
  front_pose_pred : Inport  Port=2
  rear_pose_curr : Inport  Port=3
  Bus Creator : BusCreator  Inputs=3  OutDataTypeStr=Bus: LateralBus
      settings: InheritFromInputs=off
  Constant : Constant  Value=vehicle.param.wheel_base
  Constant3 : Constant  Value=vehicle.param.max_steer_angle
  Filter steering_cmd : MATLAB Function  TreatAsAtomicUnit=on
  Plot steer command : MATLAB Function  TreatAsAtomicUnit=on
  RearToFrontOdometry : MATLAB Function  TreatAsAtomicUnit=on
  Saturate steering_cmd : MATLAB Function  TreatAsAtomicUnit=on
  Stanley controller : Subsystem
  VerifyStanleyStatus : MATLAB Function  TreatAsAtomicUnit=on
  getData : Subsystem
  is_defined_steering_tire_rotation_rate : Constant  Value=0  OutDataTypeStr=boolean
  steering_tire_rotation_rate : Constant  Value=0
  stanley_solved_status : Outport
  reason : Outport  Port=2
  ctrl_cmd : Outport  Port=3
  rear_steer : Outport  Port=4
  wires:
  ref_trajectory/1 -> getData/1(trajectory)
  front_pose_pred/1 -> getData/2(front_pose_pred)
  Constant3/1 -> Saturate steering_cmd/2(steer_limit)
  Saturate steering_cmd/1(steering_cmd_sat) -> Filter steering_cmd/1(steering_cmd_sat), Plot steer command/1(front_steer)
  Filter steering_cmd/1(steering_cmd) -> VerifyStanleyStatus/1(steering_cmd), Bus Creator/1
  steering_tire_rotation_rate/1 -> Bus Creator/2
  is_defined_steering_tire_rotation_rate/1 -> Bus Creator/3
  Bus Creator/1 -> ctrl_cmd/1
  VerifyStanleyStatus/1(stanley_solved_status) -> stanley_solved_status/1
  VerifyStanleyStatus/2(reason) -> reason/1
  getData/1(stanley_data) -> Stanley controller/1(stanley_data)
  Stanley controller/1(steering_cmd) -> Saturate steering_cmd/1(steering_cmd)
  Constant/1 -> RearToFrontOdometry/2(wheel_base)
  rear_pose_curr/1 -> RearToFrontOdometry/1(rear_pose)
  RearToFrontOdometry/1(front_pose_pred) -> getData/3(front_pose_curr)
  Stanley controller/2(rear_steer) -> rear_steer/1, Plot steer command/2(rear_steer)
